simulink model "MotorController"  (R2022b)
settings: Solver=FixedStepDiscrete  StartTime=0.0  StopTime=120  FixedStep=0.001  MaxStep=0.001  RelTol=1e-5
libraries: slpidlib x1
settings Model: Creator=szhang  LastModifiedBy=ppatel
settings SolverCC: AlgebraicLoopSolver=TrustRegion
settings DataIOCC: InitialState=simState  LimitDataPoints=on  SaveOutput=off  SaveTime=off
settings OptimizationCC: DefaultParameterBehavior=Inlined  UseDivisionForNetSlopeComputation=on  UseFloatMulNetSlope=on  InlineInvariantSignals=on  PassReuseOutputArgsAs=Individual arguments  ZeroExternalMemoryAtStartup=off  ZeroInternalMemoryAtStartup=off  NoFixptDivByZeroProtection=on  EfficientFloat2IntCast=on  LifeSpan=Inf  EfficientTunableParamExpr=on
settings DebuggingCC: SignalRangeChecking=error  SolverPrmCheckMsg=warning  IntegerOverflowMsg=error  ParameterTunabilityLossMsg=error  UnconnectedInputMsg=warning  UnconnectedOutputMsg=warning  UnconnectedLineMsg=warning  AssertControl=DisableAll  SFUnexpectedBacktrackingDiag=warning  SFNoUnconditionalDefaultTransitionDiag=warning  SFUnreachableExecutionPathDiag=error  SFExecutionAtInitializationDiag=none  SFMachineParentedDataDiag=warning  ArithmeticOperatorsInVariantConditions=warning
settings HardwareCC: ProdLongLongMode=on
settings ModelReferenceCC: EnableRefExpFcnMdlSchedulingChecks=on  PropagateSignalLabelsOutOfModel=off
settings SFSimCC: SimUseLocalCustomCode=off  MATLABDynamicMemAlloc=off  CustomCodeUndefinedFunction=UseInterfaceOnly
settings RTWCC: Description=Embedded Coder  SystemTargetFile=ert.tlc  GenCodeOnly=on  TemplateMakefile=ert_default_tmf  GenerateReport=on  RTWUseLocalCustomCode=off  IncludeHyperlinkInReport=on  PortableWordSizes=on
settings CodeAppCC: ForceParamTrailComments=on  IgnoreCustomStorageClasses=off  OperatorAnnotations=on  SimulinkDataObjDesc=on  SFDataObjDesc=on  MATLABFcnDesc=on  CustomSymbolStrGlobalVar=rt$N$M  CustomSymbolStrType=$N$M  CustomSymbolStrFcn=$N$M$F  CustomSymbolStrMacro=$N$M  InsertBlockDesc=on  StateflowObjectComments=on  MATLABSourceComments=on  ReqsInCode=on
settings ERTTargetCC: UtilityFuncGeneration=Shared location  MultiwordLength=2048  GenerateSampleERTMain=on  CombineOutputUpdateFcns=off  CombineSignalStateStructs=on  SuppressErrorStatus=on  SupportAbsoluteTime=off  SupportNonFinite=off  SupportComplex=off  ParenthesesLevel=Maximum  CastingMode=Standards  GenerateSharedConstants=off  InlinedParameterPlacement=NonHierarchical  ERTCustomFileTemplate=example_file_process.tlc  ERTFilePackagingFormat=CompactWithDataFile  EnableSignedLeftShifts=off  EnableSignedRightShifts=off
settings ConfigComp: CovEnable=on  CovScope=ReferencedModels  CovIncludeTopModel=off  CovMetricSettings=dcmw  CovHTMLOptions=-sRT=1 -sVT=0 -aTS=1 -bRG=1 -bTC=1 -hTR=0 -nFC=0 -nFD=1 -scm=1 -bcm=1 -xEv=0 -xEM=0  CovSaveCumulativeToWorkspaceVar=on  CovSaveSingleToWorkspaceVar=on  CovCumulativeReport=on  CovModelRefEnable=on  CovExternalEMLEnable=off  CovSFcnEnable=off  DVTestSuiteOptimization=CombinedObjectives (Nonlinear Extended)  DVDesignMinMaxCheck=on  DVHarnessSource=Signal Editor  PSOpenProjectManager=on  PSResultDir=ps_results_$ModelName$  PSAutoStubLUT=on
settings SimscapeCC: SimscapeNormalizeSystem=off  SimscapeLogType=all  SimscapeLogLimitData=off

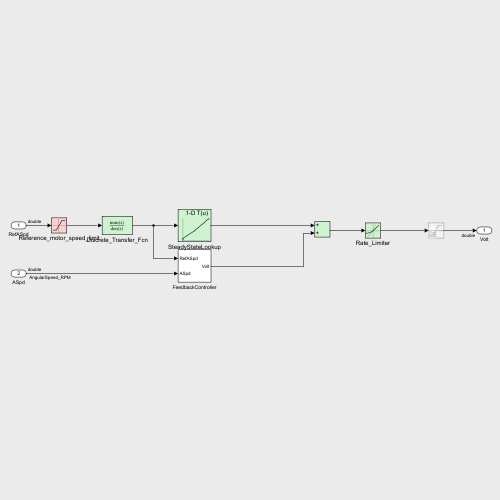
[thumbnail: Simulink's stored preview of the top-level diagram]
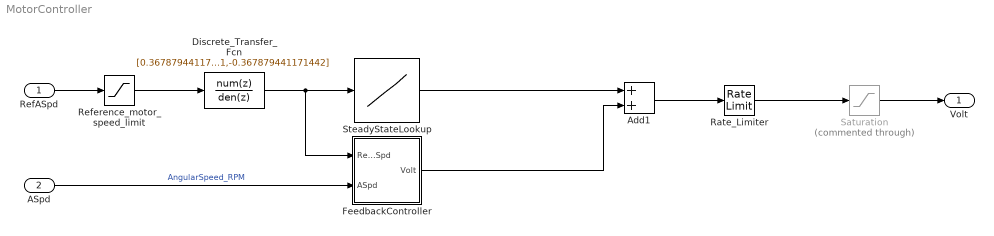
== system MotorController ==
  RefASpd : Inport  OutMin=-25000  OutMax=25000  OutDataTypeStr=double  PortDimensions=1  SampleTime=0.001
  ASpd : Inport  Port=2  OutMin=-6000  OutMax=6000  OutDataTypeStr=double  PortDimensions=1  SampleTime=0.001
  Add1 : Sum
  Discrete_Transfer_Fcn : DiscreteTransferFcn  Numerator=[0.367879441171442,0.264241117657115]  Denominator=[1,-0.367879441171442]  SampleTime=0.001
  FeedbackController : Subsystem
  Rate_Limiter : RateLimiter  RisingSlewLimit=10  FallingSlewLimit=-10  SampleTimeMode=inherited
  Reference_motor_speed_limit : Saturate  UpperLimit=5200  LowerLimit=-5200
  Saturation : Saturate  Commented=through  UpperLimit=10  LowerLimit=-10
  SteadyStateLookup : Lookup_n-D  NumberOfTableDimensions=1  BreakpointsForDimension1=[0 0.136 0.170 0.205 1.08 2.58 8.02 12.8 33.8 828.2 1535.4 2171.5 2526 3000 3827.2 4246 4775.6 4991.1 5209.4]  Table=[0 0.25 0.3 0.35 0.355 0.36 0.38 0.4 0.5 1 1.5 2 2.3 2.72 3.5 3.9 4.4 4.6 4.8]  ExtrapMethod=Clip  RemoveProtectionInput=on  UseLastTableValue=on  InternalRulePriority=Speed  RndMeth=Simplest
  Volt : Outport  OutMin=-20  OutMax=20  OutDataTypeStr=double  PortDimensions=1  SampleTime=0.001  VectorParamsAs1DForOutWhenUnconnected=off
  wires:
  ASpd/1 -> FeedbackController/2(ASpd)  "AngularSpeed_RPM"
  FeedbackController/1(Volt) -> Add1/2
  Reference_motor_speed_limit/1 -> Discrete_Transfer_Fcn/1
  Rate_Limiter/1 -> Saturation/1
  Add1/1 -> Rate_Limiter/1
  Discrete_Transfer_Fcn/1 -> FeedbackController/1(RefASpd), SteadyStateLookup/1
  SteadyStateLookup/1 -> Add1/1
  RefASpd/1 -> Reference_motor_speed_limit/1
  Saturation/1 -> Volt/1

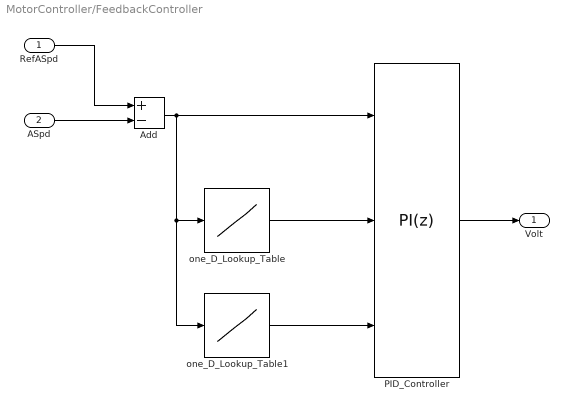
== system MotorController/FeedbackController ==
  RefASpd : Inport  OutMin=-6000  OutMax=6000
  ASpd : Inport  Port=2  OutMin=-6000  OutMax=6000
  Add : Sum  Inputs=+-
  PID_Controller : slpidlib/PID Controller  Controller=PI  Form=Parallel  TimeDomain=Discrete-time  UseExternalTs=off  SampleTime=0.001  IntegratorMethod=Forward Euler  FilterMethod=Forward Euler  ControllerParametersSource=external  P=2e-3  I=2e-3  UseKiTs=off  D=0  N=100  UseFilter=on  TunerSelectOption=Transfer Function Based (PID Tuner App)  InitialConditionSource=internal  InitialConditionForIntegrator=0  InitialConditionForFilter=0  DifferentiatorICPrevScaledInput=0  ExternalReset=none  TrackingMode=off  Kt=1  LimitOutput=on  SatLimitsSource=internal  UpperSaturationLimit=10  LowerSaturationLimit=-10  LinearizeAsGain=on  AntiWindupMode=clamping  Kb=1  LimitIntegrator=off  UpperIntegratorSaturationLimit=inf  LowerIntegratorSaturationLimit=-inf  POutMin=[]  POutMax=[]  IOutMin=[]  IOutMax=[]  DOutMin=[]  DOutMax=[]  NOutMin=[]  NOutMax=[]  SumOutMin=[]  SumOutMax=[]  SaturationOutMin=[]  SaturationOutMax=[]  PParamMin=[]  PParamMax=[]  IParamMin=[]  IParamMax=[]  DParamMin=[]  DParamMax=[]  NParamMin=[]  NParamMax=[]  KbParamMin=[]  KbParamMax=[]  KtParamMin=[]  KtParamMax=[]  KbOutMin=[]  KbOutMax=[]  KtOutMin=[]  KtOutMax=[]  IntegratorOutMin=[]  IntegratorOutMax=[]  FilterOutMin=[]  FilterOutMax=[]  SumI1OutMin=[]  SumI1OutMax=[]  SumI2OutMin=[]  SumI2OutMax=[]  SumI3OutMin=[]  SumI3OutMax=[]  SumI4OutMin=[]  SumI4OutMax=[]  SumDOutMin=[]  SumDOutMax=[]  DifferentiatorOutMin=[]  DifferentiatorOutMax=[]  FilterDiffOutCoefMin=[]  FilterDiffOutCoefMax=[]  ReciprocalOutMin=[]  ReciprocalOutMax=[]  SumDenOutMin=[]  SumDenOutMax=[]  SumNumOutMin=[]  SumNumOutMax=[]  DivideOutMin=[]  DivideOutMax=[]  UdiffTsProdOutMin=[]  UdiffTsProdOutMax=[]  NTsProdOutMin=[]  NTsProdOutMax=[]  UintegralTsProdOutMin=[]  UintegralTsProdOutMax=[]  UngainTsProdOutMin=[]  UngainTsProdOutMax=[]  ClampingZeroOutDataTypeStr=Inherit: Inherit via back propagation  ClampingZeroOutMin=[]  ClampingZeroOutMax=[]  FilterDenConstantOutDataTypeStr=Inherit: Inherit via back propagation  FilterDenConstantOutMin=[]  FilterDenConstantOutMax=[]  PCopyOutDataTypeStr=Inherit: Inherit via back propagation  PCopyOutMin=[]  PCopyOutMax=[]  NCopyOutDataTypeStr=Inherit: Inherit via back propagation  NCopyOutMin=[]  NCopyOutMax=[]  IntegratorContinuousStateAttributes=''  IntegratorStateMustResolveToSignalObject=off  IntegratorRTWStateStorageClass=Auto  FilterContinuousStateAttributes=''  FilterStateMustResolveToSignalObject=off  FilterRTWStateStorageClass=Auto  ParallelPVariant=ExternalParameters  IdealPVariant=Disabled  IVariant=ExternalParameters  DVariant=Disabled  IntegratorVariant=Discrete  SatVariant=Enabled  AWVariant=DiscClampingParallel  PCopyVariant=Disabled  TRVariant=Disabled  FdbkBlocksVariant=Forward  IdealPFdbkVariant=Disabled  SatFdbkVariant=Disabled  DerivativeFilterVariant=Disabled  NVariant=Disabled  NCopyVariant=Disabled_SignalSpec  FilterICVariant=Disabled  IntegratorICVariant=InternalICs  ExternalResetVariant=Disabled  TRSumVariant=Passthrough  SumFdbkVariant=Disabled  SumVariant=Sum_PI  TsampFilterVariant=InternalTs  TsampNgainVariant=Passthrough  TsampIntegralVariant=Passthrough  ExternalSaturationOutDataTypeStr=Inherit: Same as second input
  one_D_Lookup_Table : Lookup_n-D  NumberOfTableDimensions=1  BreakpointsForDimension1=[0 12.8 33.8 450]  Table=[1 1 1 1]*5e-4  RemoveProtectionInput=on  InternalRulePriority=Speed  RndMeth=Simplest
  one_D_Lookup_Table1 : Lookup_n-D  NumberOfTableDimensions=1  BreakpointsForDimension1=[0 12.8 33.8 450]  Table=[1 1 1 1]*5e-4  RemoveProtectionInput=on  InternalRulePriority=Speed  RndMeth=Simplest
  Volt : Outport  OutMin=-10  OutMax=10  VectorParamsAs1DForOutWhenUnconnected=off
  wires:
  ASpd/1 -> Add/2
  Add/1 -> one_D_Lookup_Table1/1, one_D_Lookup_Table/1, PID_Controller/1
  PID_Controller/1 -> Volt/1
  one_D_Lookup_Table/1 -> PID_Controller/2
  one_D_Lookup_Table1/1 -> PID_Controller/3
  RefASpd/1 -> Add/1
